simulink model "bms"  (R2025b)
settings: Solver=FixedStepAuto  StartTime=0.0  StopTime=inf  FixedStep=0.15  RelTol=1e-3
settings Model: Creator=33011  LastModifiedBy=33011

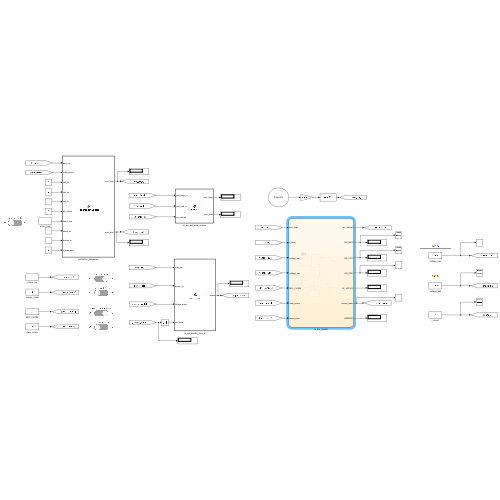
[thumbnail: Simulink's stored preview of the top-level diagram]
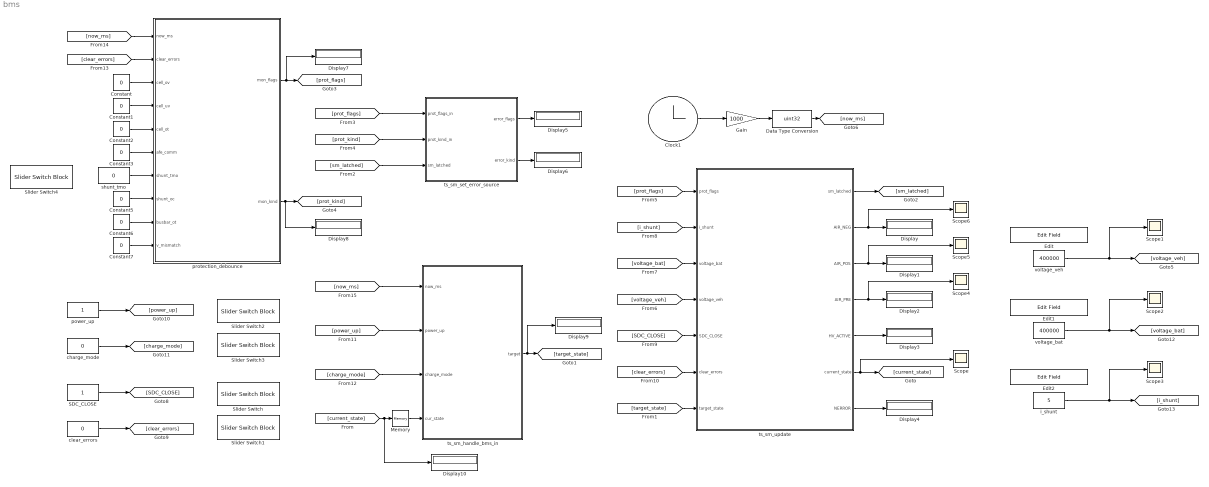
== system bms ==
  Clock1 : Clock
  Constant{,1..3,5..7} (7 alike) : Constant  Value=0
  Data Type Conversion : DataTypeConversion  OutDataTypeStr=uint32  SaturateOnIntegerOverflow=off  RndMeth=Floor
  Display{,1..10} (11 alike) : Display
  Edit : EditField  LabelPosition=Hide  ShowInitialText=on  Alignment=Center
  Edit1 : EditField  LabelPosition=Hide  ShowInitialText=on  Alignment=Center
  Edit2 : EditField  LabelPosition=Hide  ShowInitialText=on  Alignment=Center
  Gain : Gain  Gain=1000
  Memory : Memory
  SDC_CLOSE : Constant  OutDataTypeStr=uint8
  Scope{,1..6} (7 alike) : Scope
      Scope settings: ActiveDisplayYMinimum=-15.143052143259464  ActiveDisplayYMaximum=10.142564384327486
      Scope1 settings: ActiveDisplayYMinimum=-1  ActiveDisplayYMaximum=1
      Scope2 settings: ActiveDisplayYMinimum=-1  ActiveDisplayYMaximum=1  DataLoggingVariableName=ScopeData2
      Scope3 settings: ActiveDisplayYMinimum=-1  ActiveDisplayYMaximum=1  DataLoggingVariableName=ScopeData3
      Scope4 settings: ActiveDisplayYMinimum=-1  ActiveDisplayYMaximum=1  DataLoggingVariableName=ScopeData4
      Scope5 settings: ActiveDisplayYMinimum=-1  ActiveDisplayYMaximum=1  DataLoggingVariableName=ScopeData5
      Scope6 settings: ActiveDisplayYMinimum=-1  ActiveDisplayYMaximum=1  DataLoggingVariableName=ScopeData6
  Slider Switch{,1..4} (5 alike) : SliderSwitchBlock
  charge_mode : Constant  Value=0  OutDataTypeStr=uint8
  clear_errors : Constant  Value=0  OutDataTypeStr=uint8
  i_shunt : Constant  Value=5  OutDataTypeStr=int32
  power_up : Constant  OutDataTypeStr=uint8
  protection_debounce : MATLAB Function  TreatAsAtomicUnit=on
  shunt_tmo : Constant  Value=0  OutDataTypeStr=uint8
  ts_sm_handle_bms_in : MATLAB Function  TreatAsAtomicUnit=on
  ts_sm_set_error_source : MATLAB Function  TreatAsAtomicUnit=on
  ts_sm_update : Stateflow chart  TreatAsAtomicUnit=on
  voltage_bat : Constant  Value=400000  OutDataTypeStr=int32
  voltage_veh : Constant  Value=400000  OutDataTypeStr=int32
  wires:
  [power_up] -> ts_sm_handle_bms_in/2(power_up)
  [charge_mode] -> ts_sm_handle_bms_in/3(charge_mode)
  ts_sm_update/6(current_state) -> Scope/1, [current_state]
  [current_state] -> Display10/1, Memory/1
  Clock1/1 -> Gain/1
  ts_sm_handle_bms_in/1(target) -> Display9/1, [target_state]
  [target_state] -> ts_sm_update/7(target_state)
  ts_sm_update/1(sm_latched) -> [sm_latched]
  [sm_latched] -> ts_sm_set_error_source/3(sm_latched)
  ts_sm_update/2(AIR_NEG) -> Scope6/1, Display/1
  ts_sm_update/3(AIR_POS) -> Scope5/1, Display1/1
  ts_sm_update/4(AIR_PRE) -> Scope4/1, Display2/1
  ts_sm_update/5(HV_ACTIVE) -> Display3/1
  ts_sm_update/7(NERROR) -> Display4/1
  [clear_errors] -> ts_sm_update/6(clear_errors)
  [prot_flags] -> ts_sm_set_error_source/1(prot_flags_in)
  [prot_kind] -> ts_sm_set_error_source/2(prot_kind_in)
  [prot_flags] -> ts_sm_update/1(prot_flags)
  [SDC_CLOSE] -> ts_sm_update/5(SDC_CLOSE)
  [voltage_veh] -> ts_sm_update/4(voltage_veh)
  [voltage_bat] -> ts_sm_update/3(voltage_bat)
  [i_shunt] -> ts_sm_update/2(i_shunt)
  SDC_CLOSE/1 -> [SDC_CLOSE]
  clear_errors/1 -> [clear_errors]
  ts_sm_set_error_source/1(error_flags) -> Display5/1
  ts_sm_set_error_source/2(error_kind) -> Display6/1
  Memory/1 -> ts_sm_handle_bms_in/4(cur_state)
  Gain/1 -> Data Type Conversion/1
  voltage_veh/1 -> Scope1/1, [voltage_veh]
  charge_mode/1 -> [charge_mode]
  power_up/1 -> [power_up]
  voltage_bat/1 -> [voltage_bat], Scope2/1
  i_shunt/1 -> Scope3/1, [i_shunt]
  Constant/1 -> protection_debounce/3(cell_ov)
  Constant1/1 -> protection_debounce/4(cell_uv)
  Constant2/1 -> protection_debounce/5(cell_ot)
  Constant3/1 -> protection_debounce/6(afe_comm)
  shunt_tmo/1 -> protection_debounce/7(shunt_tmo)
  Constant5/1 -> protection_debounce/8(shunt_oc)
  Constant6/1 -> protection_debounce/9(busbar_ot)
  Constant7/1 -> protection_debounce/10(v_mismatch)
  [clear_errors] -> protection_debounce/2(clear_errors)
  protection_debounce/1(mon_flags) -> Display7/1, [prot_flags]
  protection_debounce/2(mon_kind) -> Display8/1, [prot_kind]
  [now_ms] -> protection_debounce/1(now_ms)
  Data Type Conversion/1 -> [now_ms]
  [now_ms] -> ts_sm_handle_bms_in/1(now_ms)

== matlab function bms/ts_sm_handle_bms_in ==
  data: now_ms input; power_up input; target output uint8; charge_mode input; cur_state input
function target = calc_target(now_ms, power_up, charge_mode, cur_state)
%#codegen
persistent t0
if isempty(t0), t0 = uint32(0); end
if power_up
    t0 = uint32(0);
    if charge_mode, target = uint8(6); else, target = uint8(1); end
elseif cur_state == uint8(1)
    if t0 == uint32(0)
        t0 = now_ms;  target = uint8(1);
    elseif uint32(now_ms) - t0 <= uint32(500)
        target = uint8(1);
    else
        t0 = uint32(0);  target = uint8(0);
    end
else
    t0 = uint32(0);  target = uint8(0);
end

== matlab function bms/ts_sm_set_error_source ==
  data: prot_flags_in input; error_flags output; prot_kind_in input; sm_latched input; error_kind output
function [error_flags, error_kind] = merge(prot_flags_in, prot_kind_in, sm_latched)
%#codegen
pf = uint16(prot_flags_in);
pk = uint16(prot_kind_in);

if sm_latched
    error_flags = bitor(pf, uint16(4));                              % bit2 状态机
    error_kind  = bitand(bitor(pk, uint16(512)), bitcmp(uint16(1))); % 512，清 NONE
else
    error_flags = pf;
    error_kind  = pk;
end

== stateflow chart bms/ts_sm_update ==
  note: 状态宏定义
      | TS_INACTIVE, //0x00
      | TS_ACTIVE, //0x01
      | TS_PRECHARGE, //0x02
      | TS_DISCHARGE, //0x03
      | TS_ERROR, //0x04
      | TS_PRE_HOLD, //0x05
      | TS_CHARGE, //0x06
  state INACTIVE
    entry:
    current_state=uint8(0);
    NERROR=uint8(1);%正常
    HV_ACTIVE=uint8(0);
    AIR_POS=uint8(0);
    AIR_NEG=uint8(0);
    AIR_PRE=uint8(0);
  note: 解锁存后且不再报错持续5s回初始状态
  note: 5s内预充失败且非故障
  state ERROR
    entry:
    current_state=uint8(4);%故障
    NERROR=uint8(0);
    HV_ACTIVE=uint8(0);
    AIR_POS=uint8(0);
    AIR_NEG=uint8(0);
    AIR_PRE=uint8(0);
  note: 目标高压或充电
  state PRECHARGE
    entry:
    current_state=uint8(2);%进预充
    HV_ACTIVE=uint8(0);
    AIR_POS=uint8(0);
    AIR_NEG=uint8(1);
    AIR_PRE=uint8(1);
  note: 清错解锁存
  note: 预充电压达到，车侧电压非零点跳动
  state PRE_HOLD
    entry:
    current_state=uint8(5);%进预充保持
    HV_ACTIVE=uint8(0);
    during:
    AIR_POS=uint8(1);
    AIR_NEG=uint8(1);
    AIR_PRE=uint8(1);
  note: 预充结束，上高压或充电
  state CHARGE
    entry:
    current_state=uint8(6);%充电状态
    HV_ACTIVE=uint8(1);
    AIR_POS=uint8(1);
    AIR_NEG=uint8(1);
    AIR_PRE=uint8(0);
  state ACTIVE
    entry:
    current_state=uint8(1);%上高压
    HV_ACTIVE=uint8(1);
    AIR_POS=uint8(1);
    AIR_NEG=uint8(1);
    AIR_PRE=uint8(0);
  note: 正常下高压放电
  state DISCHARGE
    entry:
    current_state=uint8(3);%放电状态
    HV_ACTIVE=uint8(0);
    AIR_POS=uint8(0);
    AIR_NEG=uint8(0);
    AIR_PRE=uint8(0);
  (default) -> INACTIVE : {current_state=uint8(0);%当前状态
      | AIR_POS=uint8(0);%主正继电器
      | AIR_NEG=uint8(0);%主负继电器
      | AIR_PRE=uint8(0);%预充继电器
      | HV_ACTIVE=uint8(0);%高压状态
      | sm_latched=uint8(0);%故障锁存
      | }
  (junction 112) -> INACTIVE : [duration(prot_flags==0 && sm_latched==uint8(0), sec) >= 5]{NERROR=uint8(1);}
  ERROR -> (junction 112) [order 1]
  (junction 61) -> INACTIVE
  INACTIVE -> (junction 88) [order 1] : [prot_flags != 0]
  (junction 59) -> (junction 61)
  (junction 88) -> ERROR
  INACTIVE -> PRECHARGE [order 2] : [(target_state==1||target_state==6)&&SDC_CLOSE==1]
  PRECHARGE -> ERROR [order 3] : after(5,sec)...
      | [!(voltage_veh>0.95*voltage_bat&&...
      | voltage_veh>150)&&...
      | (target_state==1||target_state==6)]{sm_latched=1;}
  PRECHARGE -> (junction 64) [order 4] : [target_state==0 || !SDC_CLOSE]
  PRECHARGE -> ERROR [order 1] : [prot_flags != 0]
  (junction 64) -> (junction 69)
  ERROR -> ERROR [order 3] : [clear_errors == 1]{sm_latched=uint8(0);}
  PRECHARGE -> PRE_HOLD [order 2] : [(voltage_veh>0.95*voltage_bat)&&...
      | (target_state==1||target_state==6)&&...
      | voltage_veh>150]
  PRE_HOLD -> ERROR [order 4] : after(200,msec)...
      | [voltage_veh <= 0.95*voltage_bat &&...
      |  (target_state==1||target_state==6)]...
      | {sm_latched=1;}
  PRE_HOLD -> (junction 69) [order 3] : [target_state==0 || !SDC_CLOSE]
  (junction 69) -> (junction 66)
  PRE_HOLD -> ERROR [order 1] : [prot_flags != 0]
  PRE_HOLD -> (junction 41) [order 2] : after(200,msec)[voltage_veh > 0.95*voltage_bat&& (target_state==1||target_state==6)]
  CHARGE -> ERROR [order 3] : [i_shunt < -300]
  (junction 41) -> ACTIVE [order 1] : [target_state==1]
  (junction 41) -> CHARGE [order 2] : [target_state==6]
  CHARGE -> ERROR [order 1] : [prot_flags != 0]
  ACTIVE -> (junction 45) [order 2] : [target_state==0||!SDC_CLOSE]
  CHARGE -> (junction 45) [order 2] : [target_state==0||!SDC_CLOSE]
  (junction 45) -> DISCHARGE
  ACTIVE -> ERROR [order 1] : [prot_flags != 0]
  (junction 103) -> ERROR
  ERROR -> (junction 54) [order 2] : [duration(prot_flags==0 && sm_latched==uint8(0), sec) >= 1]...
      | {NERROR=uint8(1);}
  DISCHARGE -> (junction 103) [order 1] : [prot_flags != 0]
  (junction 66) -> DISCHARGE
  (junction 54) -> DISCHARGE
  DISCHARGE -> (junction 59) [order 2] : after(5,sec)
  data: prot_flags input uint16; sm_latched output uint8 =0; i_shunt input int32; voltage_bat input int32; voltage_veh input int32; AIR_NEG output uint8; AIR_POS output uint8; AIR_PRE output uint8; HV_ACTIVE output uint8; current_state output uint8; SDC_CLOSE input uint8; NERROR output uint8; clear_errors input uint8; target_state input uint8

== matlab function bms/protection_debounce ==
  data: now_ms input; mon_flags output; clear_errors input; cell_ov input; mon_kind output; cell_uv input; cell_ot input; afe_comm input; shunt_tmo input; shunt_oc input; busbar_ot input; v_mismatch input
function [mon_flags, mon_kind] = error_monitor_update(now_ms, clear_errors, ...
        cell_ov, cell_uv, cell_ot, afe_comm, ...
        shunt_tmo, shunt_oc, busbar_ot, v_mismatch)
%#codegen
persistent pend conf
if isempty(pend)
    pend = zeros(1, 8, 'uint32');
    conf = false(1, 8);
end
if clear_errors
    pend = zeros(1, 8, 'uint32');
    conf = false(1, 8);
end

present = [cell_ov cell_uv cell_ot afe_comm shunt_tmo shunt_oc busbar_ot v_mismatch];
delay   = uint32([1000 1000 1000 1000 500 500 1000 1000]);
kbit    = uint16([2 4 8 256 16 32 64 128]);

for k = 1:8
    if present(k)
        if ~conf(k)
            if pend(k) == 0
                pend(k) = uint32(now_ms);
            elseif uint32(now_ms) - pend(k) >= delay(k)
                conf(k) = true;
            end
        end
    elseif ~conf(k)
        pend(k) = 0;
    end
end

mon_kind = uint16(0);
for k = 1:8
    if conf(k)
        mon_kind = bitor(mon_kind, kbit(k));
    end
end

mon_flags = uint16(0);
if any(conf(1:4)), mon_flags = bitor(mon_flags, uint16(1)); end
if any(conf(5:8)), mon_flags = bitor(mon_flags, uint16(2)); end
if mon_flags == 0
    mon_kind = uint16(1);
end
